simulink model "gm_HFMA_4B_1_5_9_13"  (R2026b)
settings: Solver=FixedStepDiscrete  StopTime=stopTime  FixedStep=1.953125e-06
PreLoadFcn:
  | load('a_luts.mat')
undefined symbols (not defined in the file or in its folder): Ts
libraries: simulink x202, simulink_need_slupdate x99, hdlsllib x91
(part 8 of 20)

== system gm_HFMA_4B_1_5_9_13/Subsystem/crp_temp_shared3 ==
  in0 : Inport  OutDataTypeStr=fixdt(1,16,15,'DataTypeOverride', 'Off')  PortDimensions=1  SampleTime=1.953125e-06
  in1 : Inport  Port=2  OutDataTypeStr=fixdt(1,16,15,'DataTypeOverride', 'Off')  PortDimensions=1  SampleTime=1.953125e-06
  in2 : Inport  Port=3  OutDataTypeStr=fixdt(1,16,15,'DataTypeOverride', 'Off')  PortDimensions=1  SampleTime=1.953125e-06
  in3 : Inport  Port=4  OutDataTypeStr=fixdt(1,16,15,'DataTypeOverride', 'Off')  PortDimensions=1  SampleTime=1.953125e-06
  in4 : Inport  Port=5  OutDataTypeStr=fixdt(1,16,15,'DataTypeOverride', 'Off')  PortDimensions=1  SampleTime=1.953125e-06
  in5 : Inport  Port=6  OutDataTypeStr=fixdt(1,16,15,'DataTypeOverride', 'Off')  PortDimensions=1  SampleTime=1.953125e-06
  in6 : Inport  Port=7  OutDataTypeStr=fixdt(1,16,15,'DataTypeOverride', 'Off')  PortDimensions=1  SampleTime=1.953125e-06
  in7 : Inport  Port=8  OutDataTypeStr=fixdt(1,16,15,'DataTypeOverride', 'Off')  PortDimensions=1  SampleTime=1.953125e-06
  in8 : Inport  Port=9  OutDataTypeStr=fixdt(1,16,15,'DataTypeOverride', 'Off')  PortDimensions=1  SampleTime=1.953125e-06
  in9 : Inport  Port=10  OutDataTypeStr=fixdt(1,16,15,'DataTypeOverride', 'Off')  PortDimensions=1  SampleTime=1.953125e-06
  in10 : Inport  Port=11  OutDataTypeStr=fixdt(1,16,15,'DataTypeOverride', 'Off')  PortDimensions=1  SampleTime=1.953125e-06
  in11 : Inport  Port=12  OutDataTypeStr=fixdt(1,16,15,'DataTypeOverride', 'Off')  PortDimensions=1  SampleTime=1.953125e-06
  in12 : Inport  Port=13  OutDataTypeStr=fixdt(1,16,15,'DataTypeOverride', 'Off')  PortDimensions=1  SampleTime=1.953125e-06
  in13 : Inport  Port=14  OutDataTypeStr=fixdt(1,16,15,'DataTypeOverride', 'Off')  PortDimensions=1  SampleTime=1.953125e-06
  in14 : Inport  Port=15  OutDataTypeStr=fixdt(1,16,15,'DataTypeOverride', 'Off')  PortDimensions=1  SampleTime=1.953125e-06
  in15 : Inport  Port=16  OutDataTypeStr=fixdt(1,16,15,'DataTypeOverride', 'Off')  PortDimensions=1  SampleTime=1.953125e-06
  enb_counter : Inport  Port=17  OutDataTypeStr=fixdt(0,6,0,'DataTypeOverride', 'Off')  PortDimensions=1  SampleTime=1.953125e-06
  Gain1 : Product  Inputs=**  OutDataTypeStr=fixdt(1, 35, 0)  SampleTime=1.953125e-06
  Gain11_const : Constant  Value=0.068999767303466796875  OutDataTypeStr=fixdt(0, 18, 21)  SampleTime=1.953125e-06
  Gain12_const : Constant  Value=0.773799896240234375  OutDataTypeStr=fixdt(0, 18, 18)  SampleTime=1.953125e-06
  Gain13_const : Constant  Value=0.068999767303466796875  OutDataTypeStr=fixdt(0, 18, 21)  SampleTime=1.953125e-06
  Gain14_const : Constant  Value=-0.1882991790771484375  OutDataTypeStr=fixdt(1, 18, 19)  SampleTime=1.953125e-06
  Gain15_const : Constant  Value=0.03100001811981201171875  OutDataTypeStr=fixdt(0, 18, 23)  SampleTime=1.953125e-06
  Gain16_const : Constant  Value=-0.107700347900390625  OutDataTypeStr=fixdt(1, 18, 20)  SampleTime=1.953125e-06
  Gain17_const : Constant  Value=-0.0090999603271484375  OutDataTypeStr=fixdt(1, 18, 23)  SampleTime=1.953125e-06
  Gain18_const : Constant  Value=-0.0370998382568359375  OutDataTypeStr=fixdt(1, 18, 21)  SampleTime=1.953125e-06
  Gain19_const : Constant  Value=-0.0220000743865966796875  OutDataTypeStr=fixdt(1, 18, 22)  SampleTime=1.953125e-06
  Gain1_const : Constant  Value=-0.003899991512298583984375  OutDataTypeStr=fixdt(1, 18, 25)  SampleTime=1.953125e-06
  Gain20_const : Constant  Value=-0.004499971866607666015625  OutDataTypeStr=fixdt(1, 18, 24)  SampleTime=1.953125e-06
  Gain21_const : Constant  Value=-0.0132000446319580078125  OutDataTypeStr=fixdt(1, 18, 23)  SampleTime=1.953125e-06
  Gain22_const : Constant  Value=0.001299999654293060302734375  OutDataTypeStr=fixdt(0, 18, 27)  SampleTime=1.953125e-06
  Gain23_const : Constant  Value=-0.003899991512298583984375  OutDataTypeStr=fixdt(1, 18, 25)  SampleTime=1.953125e-06
  Gain24_const : Constant  Value=0.0005999989807605743408203125  OutDataTypeStr=fixdt(0, 18, 28)  SampleTime=1.953125e-06
  Gain_const : Constant  Value=0.0005999989807605743408203125  OutDataTypeStr=fixdt(0, 18, 28)  SampleTime=1.953125e-06
  Serializer_Subnetwork : Subsystem
  Serializer_Subnetwork1 : Subsystem
  counter : Subsystem
  demux : Demux  Outputs=16
  enb_counter_eq_15 : simulink/Logic and Bit Operations/Compare To Constant  relop===  const=15  OutDataTypeStr=boolean
  enb_counter_le_15 : simulink/Logic and Bit Operations/Compare To Constant  relop=<=  const=15  OutDataTypeStr=boolean
  mux : Mux  Inputs=16
  mux1 : Mux  Inputs=16
  nequ_dtc{,1..15} (16 alike) : DataTypeConversion  OutDataTypeStr=fixdt(1, 19, 0)  ConvertRealWorld=Stored Integer (SI)  SampleTime=1.953125e-06  SaturateOnIntegerOverflow=off  RndMeth=Floor
  nequ_dtc{16..31} (16 alike) : DataTypeConversion  OutDataTypeStr=fixdt(1, 17, 0)  ConvertRealWorld=Stored Integer (SI)  SampleTime=1.953125e-06  SaturateOnIntegerOverflow=off  RndMeth=Floor
  nequ_dtc32 : DataTypeConversion  OutDataTypeStr=fixdt(1, 34, 40)  ConvertRealWorld=Stored Integer (SI)  SampleTime=1.953125e-06  SaturateOnIntegerOverflow=off  RndMeth=Floor
  nequ_dtc33 : DataTypeConversion  OutDataTypeStr=fixdt(1, 34, 43)  ConvertRealWorld=Stored Integer (SI)  SampleTime=1.953125e-06  SaturateOnIntegerOverflow=off  RndMeth=Floor
  nequ_dtc34 : DataTypeConversion  OutDataTypeStr=fixdt(1, 34, 43)  ConvertRealWorld=Stored Integer (SI)  SampleTime=1.953125e-06  SaturateOnIntegerOverflow=off  RndMeth=Floor
  nequ_dtc35 : DataTypeConversion  OutDataTypeStr=fixdt(1, 34, 40)  ConvertRealWorld=Stored Integer (SI)  SampleTime=1.953125e-06  SaturateOnIntegerOverflow=off  RndMeth=Floor
  nequ_dtc36 : DataTypeConversion  OutDataTypeStr=fixdt(1, 34, 42)  ConvertRealWorld=Stored Integer (SI)  SampleTime=1.953125e-06  SaturateOnIntegerOverflow=off  RndMeth=Floor
  nequ_dtc37 : DataTypeConversion  OutDataTypeStr=fixdt(1, 34, 38)  ConvertRealWorld=Stored Integer (SI)  SampleTime=1.953125e-06  SaturateOnIntegerOverflow=off  RndMeth=Floor
  nequ_dtc38 : DataTypeConversion  OutDataTypeStr=fixdt(1, 34, 39)  ConvertRealWorld=Stored Integer (SI)  SampleTime=1.953125e-06  SaturateOnIntegerOverflow=off  RndMeth=Floor
  nequ_dtc39 : DataTypeConversion  OutDataTypeStr=fixdt(1, 34, 37)  ConvertRealWorld=Stored Integer (SI)  SampleTime=1.953125e-06  SaturateOnIntegerOverflow=off  RndMeth=Floor
  nequ_dtc40 : DataTypeConversion  OutDataTypeStr=fixdt(1, 34, 36)  ConvertRealWorld=Stored Integer (SI)  SampleTime=1.953125e-06  SaturateOnIntegerOverflow=off  RndMeth=Floor
  nequ_dtc41 : DataTypeConversion  OutDataTypeStr=fixdt(1, 34, 38)  ConvertRealWorld=Stored Integer (SI)  SampleTime=1.953125e-06  SaturateOnIntegerOverflow=off  RndMeth=Floor
  nequ_dtc42 : DataTypeConversion  OutDataTypeStr=fixdt(1, 34, 35)  ConvertRealWorld=Stored Integer (SI)  SampleTime=1.953125e-06  SaturateOnIntegerOverflow=off  RndMeth=Floor
  nequ_dtc43 : DataTypeConversion  OutDataTypeStr=fixdt(1, 34, 38)  ConvertRealWorld=Stored Integer (SI)  SampleTime=1.953125e-06  SaturateOnIntegerOverflow=off  RndMeth=Floor
  nequ_dtc44 : DataTypeConversion  OutDataTypeStr=fixdt(1, 34, 34)  ConvertRealWorld=Stored Integer (SI)  SampleTime=1.953125e-06  SaturateOnIntegerOverflow=off  RndMeth=Floor
  nequ_dtc45 : DataTypeConversion  OutDataTypeStr=fixdt(1, 34, 36)  ConvertRealWorld=Stored Integer (SI)  SampleTime=1.953125e-06  SaturateOnIntegerOverflow=off  RndMeth=Floor
  nequ_dtc46 : DataTypeConversion  OutDataTypeStr=fixdt(1, 34, 33)  ConvertRealWorld=Stored Integer (SI)  SampleTime=1.953125e-06  SaturateOnIntegerOverflow=off  RndMeth=Floor
  nequ_dtc47 : DataTypeConversion  OutDataTypeStr=fixdt(1, 34, 36)  ConvertRealWorld=Stored Integer (SI)  SampleTime=1.953125e-06  SaturateOnIntegerOverflow=off  RndMeth=Floor
  tapped_delay : hdlsllib/Discrete/Tapped Delay Enabled Synchronous  vinit=0  samptime=-1  NumDelays=15  DelayOrder=Oldest  includeCurrent=on
  tapped_delay_outunit_delay : simulink_need_slupdate/Unit Delay Enabled  vinit=0.0  tsamp=-1
  out0 : Outport  OutDataTypeStr=fixdt(1,34,40,'DataTypeOverride', 'Off')  PortDimensions=1  SampleTime=1.953125e-06
  out1 : Outport  Port=2  OutDataTypeStr=fixdt(1,34,43,'DataTypeOverride', 'Off')  PortDimensions=1  SampleTime=1.953125e-06
  out2 : Outport  Port=3  OutDataTypeStr=fixdt(1,34,43,'DataTypeOverride', 'Off')  PortDimensions=1  SampleTime=1.953125e-06
  out3 : Outport  Port=4  OutDataTypeStr=fixdt(1,34,40,'DataTypeOverride', 'Off')  PortDimensions=1  SampleTime=1.953125e-06
  out4 : Outport  Port=5  OutDataTypeStr=fixdt(1,34,42,'DataTypeOverride', 'Off')  PortDimensions=1  SampleTime=1.953125e-06
  out5 : Outport  Port=6  OutDataTypeStr=fixdt(1,34,38,'DataTypeOverride', 'Off')  PortDimensions=1  SampleTime=1.953125e-06
  out6 : Outport  Port=7  OutDataTypeStr=fixdt(1,34,39,'DataTypeOverride', 'Off')  PortDimensions=1  SampleTime=1.953125e-06
  out7 : Outport  Port=8  OutDataTypeStr=fixdt(1,34,37,'DataTypeOverride', 'Off')  PortDimensions=1  SampleTime=1.953125e-06
  out8 : Outport  Port=9  OutDataTypeStr=fixdt(1,34,36,'DataTypeOverride', 'Off')  PortDimensions=1  SampleTime=1.953125e-06
  out9 : Outport  Port=10  OutDataTypeStr=fixdt(1,34,38,'DataTypeOverride', 'Off')  PortDimensions=1  SampleTime=1.953125e-06
  out10 : Outport  Port=11  OutDataTypeStr=fixdt(1,34,35,'DataTypeOverride', 'Off')  PortDimensions=1  SampleTime=1.953125e-06
  out11 : Outport  Port=12  OutDataTypeStr=fixdt(1,34,38,'DataTypeOverride', 'Off')  PortDimensions=1  SampleTime=1.953125e-06
  out12 : Outport  Port=13  OutDataTypeStr=fixdt(1,34,34,'DataTypeOverride', 'Off')  PortDimensions=1  SampleTime=1.953125e-06
  out13 : Outport  Port=14  OutDataTypeStr=fixdt(1,34,36,'DataTypeOverride', 'Off')  PortDimensions=1  SampleTime=1.953125e-06
  out14 : Outport  Port=15  OutDataTypeStr=fixdt(1,34,33,'DataTypeOverride', 'Off')  PortDimensions=1  SampleTime=1.953125e-06
  out15 : Outport  Port=16  OutDataTypeStr=fixdt(1,34,36,'DataTypeOverride', 'Off')  PortDimensions=1  SampleTime=1.953125e-06
  wires:
  Gain_const/1 -> nequ_dtc1/1
  Gain1/1 -> tapped_delay/1
  Gain23_const/1 -> nequ_dtc3/1
  nequ_dtc47/1 -> out15/1
  Gain1_const/1 -> nequ_dtc/1
  Gain24_const/1 -> nequ_dtc2/1
  nequ_dtc18/1 -> mux1/3
  Gain22_const/1 -> nequ_dtc4/1
  Gain20_const/1 -> nequ_dtc6/1
  Gain21_const/1 -> nequ_dtc5/1
  Gain13_const/1 -> nequ_dtc13/1
  Gain15_const/1 -> nequ_dtc11/1
  Gain17_const/1 -> nequ_dtc9/1
  Gain19_const/1 -> nequ_dtc7/1
  Gain12_const/1 -> nequ_dtc14/1
  Gain14_const/1 -> nequ_dtc12/1
  Gain16_const/1 -> nequ_dtc10/1
  Gain18_const/1 -> nequ_dtc8/1
  Gain11_const/1 -> nequ_dtc15/1
  nequ_dtc42/1 -> out10/1
  in0/1 -> nequ_dtc16/1
  nequ_dtc43/1 -> out11/1
  in1/1 -> nequ_dtc17/1
  in6/1 -> nequ_dtc22/1
  in2/1 -> nequ_dtc18/1
  in3/1 -> nequ_dtc19/1
  in4/1 -> nequ_dtc20/1
  nequ_dtc39/1 -> out7/1
  in5/1 -> nequ_dtc21/1
  in11/1 -> nequ_dtc27/1
  in7/1 -> nequ_dtc23/1
  demux/13 -> nequ_dtc44/1
  in12/1 -> nequ_dtc28/1
  demux/9 -> nequ_dtc40/1
  in8/1 -> nequ_dtc24/1
  demux/12 -> nequ_dtc43/1
  in9/1 -> nequ_dtc25/1
  in10/1 -> nequ_dtc26/1
  in13/1 -> nequ_dtc29/1
  nequ_dtc30/1 -> mux1/15
  demux/7 -> nequ_dtc38/1
  in14/1 -> nequ_dtc30/1
  in15/1 -> nequ_dtc31/1
  demux/1 -> nequ_dtc32/1
  enb_counter/1 -> enb_counter_eq_15/1, enb_counter_le_15/1
  nequ_dtc/1 -> mux/1
  nequ_dtc1/1 -> mux/2
  nequ_dtc2/1 -> mux/3
  nequ_dtc3/1 -> mux/4
  nequ_dtc8/1 -> mux/9
  nequ_dtc4/1 -> mux/5
  nequ_dtc5/1 -> mux/6
  nequ_dtc6/1 -> mux/7
  nequ_dtc7/1 -> mux/8
  nequ_dtc13/1 -> mux/14
  nequ_dtc9/1 -> mux/10
  nequ_dtc10/1 -> mux/11
  nequ_dtc11/1 -> mux/12
  nequ_dtc12/1 -> mux/13
  nequ_dtc14/1 -> mux/15
  nequ_dtc15/1 -> mux/16
  nequ_dtc16/1 -> mux1/1
  nequ_dtc17/1 -> mux1/2
  nequ_dtc23/1 -> mux1/8
  nequ_dtc19/1 -> mux1/4
  nequ_dtc20/1 -> mux1/5
  nequ_dtc21/1 -> mux1/6
  nequ_dtc22/1 -> mux1/7
  nequ_dtc28/1 -> mux1/13
  nequ_dtc24/1 -> mux1/9
  nequ_dtc29/1 -> mux1/14
  nequ_dtc25/1 -> mux1/10
  nequ_dtc26/1 -> mux1/11
  nequ_dtc27/1 -> mux1/12
  nequ_dtc31/1 -> mux1/16
  enb_counter_le_15/1 -> counter/Enable, tapped_delay/2
  mux/1 -> Serializer_Subnetwork/1(in0)
  mux1/1 -> Serializer_Subnetwork1/1(in0)
  counter/1(out0) -> Serializer_Subnetwork1/2(in1), Serializer_Subnetwork/2(in1)
  Serializer_Subnetwork/1(out0) -> Gain1/1
  demux/2 -> nequ_dtc33/1
  Serializer_Subnetwork1/1(out0) -> Gain1/2
  enb_counter_eq_15/1 -> tapped_delay_outunit_delay/2
  tapped_delay/1 -> tapped_delay_outunit_delay/1
  tapped_delay_outunit_delay/1 -> demux/1
  demux/3 -> nequ_dtc34/1
  demux/4 -> nequ_dtc35/1
  demux/5 -> nequ_dtc36/1
  demux/6 -> nequ_dtc37/1
  demux/8 -> nequ_dtc39/1
  demux/10 -> nequ_dtc41/1
  demux/11 -> nequ_dtc42/1
  demux/14 -> nequ_dtc45/1
  demux/15 -> nequ_dtc46/1
  demux/16 -> nequ_dtc47/1
  nequ_dtc32/1 -> out0/1
  nequ_dtc33/1 -> out1/1
  nequ_dtc34/1 -> out2/1
  nequ_dtc35/1 -> out3/1
  nequ_dtc36/1 -> out4/1
  nequ_dtc37/1 -> out5/1
  nequ_dtc38/1 -> out6/1
  nequ_dtc40/1 -> out8/1
  nequ_dtc41/1 -> out9/1
  nequ_dtc44/1 -> out12/1
  nequ_dtc45/1 -> out13/1
  nequ_dtc46/1 -> out14/1

== system gm_HFMA_4B_1_5_9_13/Subsystem/crp_temp_shared4 ==
  in0 : Inport  OutDataTypeStr=fixdt(1,16,15,'DataTypeOverride', 'Off')  PortDimensions=1  SampleTime=1.953125e-06
  in1 : Inport  Port=2  OutDataTypeStr=fixdt(1,16,15,'DataTypeOverride', 'Off')  PortDimensions=1  SampleTime=1.953125e-06
  in2 : Inport  Port=3  OutDataTypeStr=fixdt(1,16,15,'DataTypeOverride', 'Off')  PortDimensions=1  SampleTime=1.953125e-06
  in3 : Inport  Port=4  OutDataTypeStr=fixdt(1,16,15,'DataTypeOverride', 'Off')  PortDimensions=1  SampleTime=1.953125e-06
  in4 : Inport  Port=5  OutDataTypeStr=fixdt(1,16,15,'DataTypeOverride', 'Off')  PortDimensions=1  SampleTime=1.953125e-06
  in5 : Inport  Port=6  OutDataTypeStr=fixdt(1,16,15,'DataTypeOverride', 'Off')  PortDimensions=1  SampleTime=1.953125e-06
  in6 : Inport  Port=7  OutDataTypeStr=fixdt(1,16,15,'DataTypeOverride', 'Off')  PortDimensions=1  SampleTime=1.953125e-06
  in7 : Inport  Port=8  OutDataTypeStr=fixdt(1,16,15,'DataTypeOverride', 'Off')  PortDimensions=1  SampleTime=1.953125e-06
  in8 : Inport  Port=9  OutDataTypeStr=fixdt(1,16,15,'DataTypeOverride', 'Off')  PortDimensions=1  SampleTime=1.953125e-06
  in9 : Inport  Port=10  OutDataTypeStr=fixdt(1,16,15,'DataTypeOverride', 'Off')  PortDimensions=1  SampleTime=1.953125e-06
  in10 : Inport  Port=11  OutDataTypeStr=fixdt(1,16,15,'DataTypeOverride', 'Off')  PortDimensions=1  SampleTime=1.953125e-06
  in11 : Inport  Port=12  OutDataTypeStr=fixdt(1,16,15,'DataTypeOverride', 'Off')  PortDimensions=1  SampleTime=1.953125e-06
  in12 : Inport  Port=13  OutDataTypeStr=fixdt(1,16,15,'DataTypeOverride', 'Off')  PortDimensions=1  SampleTime=1.953125e-06
  in13 : Inport  Port=14  OutDataTypeStr=fixdt(1,16,15,'DataTypeOverride', 'Off')  PortDimensions=1  SampleTime=1.953125e-06
  in14 : Inport  Port=15  OutDataTypeStr=fixdt(1,16,15,'DataTypeOverride', 'Off')  PortDimensions=1  SampleTime=1.953125e-06
  in15 : Inport  Port=16  OutDataTypeStr=fixdt(1,16,15,'DataTypeOverride', 'Off')  PortDimensions=1  SampleTime=1.953125e-06
  enb_counter : Inport  Port=17  OutDataTypeStr=fixdt(0,6,0,'DataTypeOverride', 'Off')  PortDimensions=1  SampleTime=1.953125e-06
  Gain10 : Product  Inputs=**  OutDataTypeStr=fixdt(1, 35, 0)  SampleTime=1.953125e-06
  Gain10_const : Constant  Value=-0.1882991790771484375  OutDataTypeStr=fixdt(1, 18, 19)  SampleTime=1.953125e-06
  Gain1_const : Constant  Value=-0.003899991512298583984375  OutDataTypeStr=fixdt(1, 18, 25)  SampleTime=1.953125e-06
  Gain20_const : Constant  Value=-0.004499971866607666015625  OutDataTypeStr=fixdt(1, 18, 24)  SampleTime=1.953125e-06
  Gain21_const : Constant  Value=-0.0132000446319580078125  OutDataTypeStr=fixdt(1, 18, 23)  SampleTime=1.953125e-06
  Gain22_const : Constant  Value=0.001299999654293060302734375  OutDataTypeStr=fixdt(0, 18, 27)  SampleTime=1.953125e-06
  Gain23_const : Constant  Value=-0.003899991512298583984375  OutDataTypeStr=fixdt(1, 18, 25)  SampleTime=1.953125e-06
  Gain24_const : Constant  Value=0.0005999989807605743408203125  OutDataTypeStr=fixdt(0, 18, 28)  SampleTime=1.953125e-06
  Gain2_const : Constant  Value=0.001299999654293060302734375  OutDataTypeStr=fixdt(0, 18, 27)  SampleTime=1.953125e-06
  Gain3_const : Constant  Value=-0.0132000446319580078125  OutDataTypeStr=fixdt(1, 18, 23)  SampleTime=1.953125e-06
  Gain4_const : Constant  Value=-0.004499971866607666015625  OutDataTypeStr=fixdt(1, 18, 24)  SampleTime=1.953125e-06
  Gain5_const : Constant  Value=-0.0220000743865966796875  OutDataTypeStr=fixdt(1, 18, 22)  SampleTime=1.953125e-06
  Gain6_const : Constant  Value=-0.0370998382568359375  OutDataTypeStr=fixdt(1, 18, 21)  SampleTime=1.953125e-06
  Gain7_const : Constant  Value=-0.0090999603271484375  OutDataTypeStr=fixdt(1, 18, 23)  SampleTime=1.953125e-06
  Gain8_const : Constant  Value=-0.107700347900390625  OutDataTypeStr=fixdt(1, 18, 20)  SampleTime=1.953125e-06
  Gain9_const : Constant  Value=0.03100001811981201171875  OutDataTypeStr=fixdt(0, 18, 23)  SampleTime=1.953125e-06
  Gain_const : Constant  Value=0.0005999989807605743408203125  OutDataTypeStr=fixdt(0, 18, 28)  SampleTime=1.953125e-06
  Serializer_Subnetwork : Subsystem
  Serializer_Subnetwork1 : Subsystem
  counter : Subsystem
  demux : Demux  Outputs=16
  enb_counter_eq_15 : simulink/Logic and Bit Operations/Compare To Constant  relop===  const=15  OutDataTypeStr=boolean
  enb_counter_le_15 : simulink/Logic and Bit Operations/Compare To Constant  relop=<=  const=15  OutDataTypeStr=boolean
  mux : Mux  Inputs=16
  mux1 : Mux  Inputs=16
  nequ_dtc{,1..15} (16 alike) : DataTypeConversion  OutDataTypeStr=fixdt(1, 19, 0)  ConvertRealWorld=Stored Integer (SI)  SampleTime=1.953125e-06  SaturateOnIntegerOverflow=off  RndMeth=Floor
  nequ_dtc{16..31} (16 alike) : DataTypeConversion  OutDataTypeStr=fixdt(1, 17, 0)  ConvertRealWorld=Stored Integer (SI)  SampleTime=1.953125e-06  SaturateOnIntegerOverflow=off  RndMeth=Floor
  nequ_dtc32 : DataTypeConversion  OutDataTypeStr=fixdt(1, 34, 34)  ConvertRealWorld=Stored Integer (SI)  SampleTime=1.953125e-06  SaturateOnIntegerOverflow=off  RndMeth=Floor
  nequ_dtc{33,35,39,46} (4 alike) : DataTypeConversion  OutDataTypeStr=fixdt(1, 34, 38)  ConvertRealWorld=Stored Integer (SI)  SampleTime=1.953125e-06  SaturateOnIntegerOverflow=off  RndMeth=Floor
  nequ_dtc34 : DataTypeConversion  OutDataTypeStr=fixdt(1, 34, 35)  ConvertRealWorld=Stored Integer (SI)  SampleTime=1.953125e-06  SaturateOnIntegerOverflow=off  RndMeth=Floor
  nequ_dtc36 : DataTypeConversion  OutDataTypeStr=fixdt(1, 34, 36)  ConvertRealWorld=Stored Integer (SI)  SampleTime=1.953125e-06  SaturateOnIntegerOverflow=off  RndMeth=Floor
  nequ_dtc37 : DataTypeConversion  OutDataTypeStr=fixdt(1, 34, 37)  ConvertRealWorld=Stored Integer (SI)  SampleTime=1.953125e-06  SaturateOnIntegerOverflow=off  RndMeth=Floor
  nequ_dtc38 : DataTypeConversion  OutDataTypeStr=fixdt(1, 34, 39)  ConvertRealWorld=Stored Integer (SI)  SampleTime=1.953125e-06  SaturateOnIntegerOverflow=off  RndMeth=Floor
  nequ_dtc40 : DataTypeConversion  OutDataTypeStr=fixdt(1, 34, 42)  ConvertRealWorld=Stored Integer (SI)  SampleTime=1.953125e-06  SaturateOnIntegerOverflow=off  RndMeth=Floor
  nequ_dtc41 : DataTypeConversion  OutDataTypeStr=fixdt(1, 34, 40)  ConvertRealWorld=Stored Integer (SI)  SampleTime=1.953125e-06  SaturateOnIntegerOverflow=off  RndMeth=Floor
  nequ_dtc42 : DataTypeConversion  OutDataTypeStr=fixdt(1, 34, 43)  ConvertRealWorld=Stored Integer (SI)  SampleTime=1.953125e-06  SaturateOnIntegerOverflow=off  RndMeth=Floor
  nequ_dtc43 : DataTypeConversion  OutDataTypeStr=fixdt(1, 34, 43)  ConvertRealWorld=Stored Integer (SI)  SampleTime=1.953125e-06  SaturateOnIntegerOverflow=off  RndMeth=Floor
  nequ_dtc44 : DataTypeConversion  OutDataTypeStr=fixdt(1, 34, 40)  ConvertRealWorld=Stored Integer (SI)  SampleTime=1.953125e-06  SaturateOnIntegerOverflow=off  RndMeth=Floor
  nequ_dtc45 : DataTypeConversion  OutDataTypeStr=fixdt(1, 34, 42)  ConvertRealWorld=Stored Integer (SI)  SampleTime=1.953125e-06  SaturateOnIntegerOverflow=off  RndMeth=Floor
  nequ_dtc47 : DataTypeConversion  OutDataTypeStr=fixdt(1, 34, 39)  ConvertRealWorld=Stored Integer (SI)  SampleTime=1.953125e-06  SaturateOnIntegerOverflow=off  RndMeth=Floor
  tapped_delay : hdlsllib/Discrete/Tapped Delay Enabled Synchronous  vinit=0  samptime=-1  NumDelays=15  DelayOrder=Oldest  includeCurrent=on
  tapped_delay_outunit_delay : simulink_need_slupdate/Unit Delay Enabled  vinit=0.0  tsamp=-1
  out0 : Outport  OutDataTypeStr=fixdt(1,34,34,'DataTypeOverride', 'Off')  PortDimensions=1  SampleTime=1.953125e-06
  out1 : Outport  Port=2  OutDataTypeStr=fixdt(1,34,38,'DataTypeOverride', 'Off')  PortDimensions=1  SampleTime=1.953125e-06
  out2 : Outport  Port=3  OutDataTypeStr=fixdt(1,34,35,'DataTypeOverride', 'Off')  PortDimensions=1  SampleTime=1.953125e-06
  out3 : Outport  Port=4  OutDataTypeStr=fixdt(1,34,38,'DataTypeOverride', 'Off')  PortDimensions=1  SampleTime=1.953125e-06
  out4 : Outport  Port=5  OutDataTypeStr=fixdt(1,34,36,'DataTypeOverride', 'Off')  PortDimensions=1  SampleTime=1.953125e-06
  out5 : Outport  Port=6  OutDataTypeStr=fixdt(1,34,37,'DataTypeOverride', 'Off')  PortDimensions=1  SampleTime=1.953125e-06
  out6 : Outport  Port=7  OutDataTypeStr=fixdt(1,34,39,'DataTypeOverride', 'Off')  PortDimensions=1  SampleTime=1.953125e-06
  out7 : Outport  Port=8  OutDataTypeStr=fixdt(1,34,38,'DataTypeOverride', 'Off')  PortDimensions=1  SampleTime=1.953125e-06
  out8 : Outport  Port=9  OutDataTypeStr=fixdt(1,34,42,'DataTypeOverride', 'Off')  PortDimensions=1  SampleTime=1.953125e-06
  out9 : Outport  Port=10  OutDataTypeStr=fixdt(1,34,40,'DataTypeOverride', 'Off')  PortDimensions=1  SampleTime=1.953125e-06
  out10 : Outport  Port=11  OutDataTypeStr=fixdt(1,34,43,'DataTypeOverride', 'Off')  PortDimensions=1  SampleTime=1.953125e-06
  out11 : Outport  Port=12  OutDataTypeStr=fixdt(1,34,43,'DataTypeOverride', 'Off')  PortDimensions=1  SampleTime=1.953125e-06
  out12 : Outport  Port=13  OutDataTypeStr=fixdt(1,34,40,'DataTypeOverride', 'Off')  PortDimensions=1  SampleTime=1.953125e-06
  out13 : Outport  Port=14  OutDataTypeStr=fixdt(1,34,42,'DataTypeOverride', 'Off')  PortDimensions=1  SampleTime=1.953125e-06
  out14 : Outport  Port=15  OutDataTypeStr=fixdt(1,34,38,'DataTypeOverride', 'Off')  PortDimensions=1  SampleTime=1.953125e-06
  out15 : Outport  Port=16  OutDataTypeStr=fixdt(1,34,39,'DataTypeOverride', 'Off')  PortDimensions=1  SampleTime=1.953125e-06
  wires:
  Gain6_const/1 -> nequ_dtc4/1
  nequ_dtc30/1 -> mux1/15
  Gain9_const/1 -> nequ_dtc1/1
  Gain10/1 -> tapped_delay/1
  Gain7_const/1 -> nequ_dtc3/1
  Gain10_const/1 -> nequ_dtc/1
  Gain8_const/1 -> nequ_dtc2/1
  Gain24_const/1 -> nequ_dtc11/1
  Gain1_const/1 -> nequ_dtc9/1
  Gain5_const/1 -> nequ_dtc5/1
  Gain3_const/1 -> nequ_dtc7/1
  Gain_const/1 -> nequ_dtc10/1
  Gain2_const/1 -> nequ_dtc8/1
  Gain4_const/1 -> nequ_dtc6/1
  Gain21_const/1 -> nequ_dtc14/1
  Gain23_const/1 -> nequ_dtc12/1
  Gain20_const/1 -> nequ_dtc15/1
  Gain22_const/1 -> nequ_dtc13/1
  nequ_dtc19/1 -> mux1/4
  in4/1 -> nequ_dtc20/1
  in0/1 -> nequ_dtc16/1
  in5/1 -> nequ_dtc21/1
  nequ_dtc22/1 -> mux1/7
  nequ_dtc18/1 -> mux1/3
  in1/1 -> nequ_dtc17/1
  nequ_dtc21/1 -> mux1/6
  nequ_dtc17/1 -> mux1/2
  in2/1 -> nequ_dtc18/1
  nequ_dtc20/1 -> mux1/5
  in3/1 -> nequ_dtc19/1
  in10/1 -> nequ_dtc26/1
  in6/1 -> nequ_dtc22/1
  in7/1 -> nequ_dtc23/1
  in8/1 -> nequ_dtc24/1
  in9/1 -> nequ_dtc25/1
  in15/1 -> nequ_dtc31/1
  in11/1 -> nequ_dtc27/1
  in12/1 -> nequ_dtc28/1
  in13/1 -> nequ_dtc29/1
  in14/1 -> nequ_dtc30/1
  enb_counter/1 -> enb_counter_eq_15/1, enb_counter_le_15/1
  nequ_dtc/1 -> mux/1
  nequ_dtc1/1 -> mux/2
  nequ_dtc6/1 -> mux/7
  nequ_dtc2/1 -> mux/3
  nequ_dtc3/1 -> mux/4
  nequ_dtc4/1 -> mux/5
  nequ_dtc5/1 -> mux/6
  nequ_dtc11/1 -> mux/12
  nequ_dtc7/1 -> mux/8
  nequ_dtc12/1 -> mux/13
  nequ_dtc8/1 -> mux/9
  nequ_dtc9/1 -> mux/10
  nequ_dtc10/1 -> mux/11
  nequ_dtc13/1 -> mux/14
  nequ_dtc14/1 -> mux/15
  nequ_dtc15/1 -> mux/16
  nequ_dtc16/1 -> mux1/1
  nequ_dtc27/1 -> mux1/12
  nequ_dtc23/1 -> mux1/8
  nequ_dtc24/1 -> mux1/9
  nequ_dtc25/1 -> mux1/10
  nequ_dtc26/1 -> mux1/11
  nequ_dtc28/1 -> mux1/13
  nequ_dtc29/1 -> mux1/14
  nequ_dtc31/1 -> mux1/16
  enb_counter_le_15/1 -> counter/Enable, tapped_delay/2
  mux/1 -> Serializer_Subnetwork/1(in0)
  mux1/1 -> Serializer_Subnetwork1/1(in0)
  counter/1(out0) -> Serializer_Subnetwork1/2(in1), Serializer_Subnetwork/2(in1)
  Serializer_Subnetwork/1(out0) -> Gain10/1
  Serializer_Subnetwork1/1(out0) -> Gain10/2
  enb_counter_eq_15/1 -> tapped_delay_outunit_delay/2
  tapped_delay/1 -> tapped_delay_outunit_delay/1
  tapped_delay_outunit_delay/1 -> demux/1
  demux/1 -> nequ_dtc32/1
  demux/2 -> nequ_dtc33/1
  demux/3 -> nequ_dtc34/1
  demux/4 -> nequ_dtc35/1
  demux/5 -> nequ_dtc36/1
  demux/6 -> nequ_dtc37/1
  demux/7 -> nequ_dtc38/1
  demux/8 -> nequ_dtc39/1
  demux/9 -> nequ_dtc40/1
  demux/10 -> nequ_dtc41/1
  demux/11 -> nequ_dtc42/1
  demux/12 -> nequ_dtc43/1
  demux/13 -> nequ_dtc44/1
  demux/14 -> nequ_dtc45/1
  demux/15 -> nequ_dtc46/1
  demux/16 -> nequ_dtc47/1
  nequ_dtc32/1 -> out0/1
  nequ_dtc33/1 -> out1/1
  nequ_dtc34/1 -> out2/1
  nequ_dtc35/1 -> out3/1
  nequ_dtc36/1 -> out4/1
  nequ_dtc37/1 -> out5/1
  nequ_dtc38/1 -> out6/1
  nequ_dtc39/1 -> out7/1
  nequ_dtc40/1 -> out8/1
  nequ_dtc41/1 -> out9/1
  nequ_dtc42/1 -> out10/1
  nequ_dtc43/1 -> out11/1
  nequ_dtc44/1 -> out12/1
  nequ_dtc45/1 -> out13/1
  nequ_dtc46/1 -> out14/1
  nequ_dtc47/1 -> out15/1

== system gm_HFMA_4B_1_5_9_13/Subsystem/crp_temp_shared5 ==
  in0 : Inport  OutDataTypeStr=fixdt(1,16,15,'DataTypeOverride', 'Off')  PortDimensions=1  SampleTime=1.953125e-06
  in1 : Inport  Port=2  OutDataTypeStr=fixdt(1,16,15,'DataTypeOverride', 'Off')  PortDimensions=1  SampleTime=1.953125e-06
  in2 : Inport  Port=3  OutDataTypeStr=fixdt(1,16,15,'DataTypeOverride', 'Off')  PortDimensions=1  SampleTime=1.953125e-06
  in3 : Inport  Port=4  OutDataTypeStr=fixdt(1,16,15,'DataTypeOverride', 'Off')  PortDimensions=1  SampleTime=1.953125e-06
  in4 : Inport  Port=5  OutDataTypeStr=fixdt(1,16,15,'DataTypeOverride', 'Off')  PortDimensions=1  SampleTime=1.953125e-06
  in5 : Inport  Port=6  OutDataTypeStr=fixdt(1,16,15,'DataTypeOverride', 'Off')  PortDimensions=1  SampleTime=1.953125e-06
  in6 : Inport  Port=7  OutDataTypeStr=fixdt(1,16,15,'DataTypeOverride', 'Off')  PortDimensions=1  SampleTime=1.953125e-06
  in7 : Inport  Port=8  OutDataTypeStr=fixdt(1,16,15,'DataTypeOverride', 'Off')  PortDimensions=1  SampleTime=1.953125e-06
  in8 : Inport  Port=9  OutDataTypeStr=fixdt(1,16,15,'DataTypeOverride', 'Off')  PortDimensions=1  SampleTime=1.953125e-06
  in9 : Inport  Port=10  OutDataTypeStr=fixdt(1,16,15,'DataTypeOverride', 'Off')  PortDimensions=1  SampleTime=1.953125e-06
  in10 : Inport  Port=11  OutDataTypeStr=fixdt(1,16,15,'DataTypeOverride', 'Off')  PortDimensions=1  SampleTime=1.953125e-06
  in11 : Inport  Port=12  OutDataTypeStr=fixdt(1,16,15,'DataTypeOverride', 'Off')  PortDimensions=1  SampleTime=1.953125e-06
  in12 : Inport  Port=13  OutDataTypeStr=fixdt(1,16,15,'DataTypeOverride', 'Off')  PortDimensions=1  SampleTime=1.953125e-06
  in13 : Inport  Port=14  OutDataTypeStr=fixdt(1,16,15,'DataTypeOverride', 'Off')  PortDimensions=1  SampleTime=1.953125e-06
  in14 : Inport  Port=15  OutDataTypeStr=fixdt(1,16,15,'DataTypeOverride', 'Off')  PortDimensions=1  SampleTime=1.953125e-06
  in15 : Inport  Port=16  OutDataTypeStr=fixdt(1,16,15,'DataTypeOverride', 'Off')  PortDimensions=1  SampleTime=1.953125e-06
  enb_counter : Inport  Port=17  OutDataTypeStr=fixdt(0,6,0,'DataTypeOverride', 'Off')  PortDimensions=1  SampleTime=1.953125e-06
  Gain10_const : Constant  Value=-0.1882991790771484375  OutDataTypeStr=fixdt(1, 18, 19)  SampleTime=1.953125e-06
  Gain11_const : Constant  Value=0.068999767303466796875  OutDataTypeStr=fixdt(0, 18, 21)  SampleTime=1.953125e-06
  Gain12_const : Constant  Value=0.773799896240234375  OutDataTypeStr=fixdt(0, 18, 18)  SampleTime=1.953125e-06
  Gain13_const : Constant  Value=0.068999767303466796875  OutDataTypeStr=fixdt(0, 18, 21)  SampleTime=1.953125e-06
  Gain14_const : Constant  Value=-0.1882991790771484375  OutDataTypeStr=fixdt(1, 18, 19)  SampleTime=1.953125e-06
  Gain15_const : Constant  Value=0.03100001811981201171875  OutDataTypeStr=fixdt(0, 18, 23)  SampleTime=1.953125e-06
  Gain16_const : Constant  Value=-0.107700347900390625  OutDataTypeStr=fixdt(1, 18, 20)  SampleTime=1.953125e-06
  Gain17_const : Constant  Value=-0.0090999603271484375  OutDataTypeStr=fixdt(1, 18, 23)  SampleTime=1.953125e-06
  Gain18_const : Constant  Value=-0.0370998382568359375  OutDataTypeStr=fixdt(1, 18, 21)  SampleTime=1.953125e-06
  Gain19 : Product  Inputs=**  OutDataTypeStr=fixdt(1, 35, 0)  SampleTime=1.953125e-06
  Gain19_const : Constant  Value=-0.0220000743865966796875  OutDataTypeStr=fixdt(1, 18, 22)  SampleTime=1.953125e-06
  Gain4_const : Constant  Value=-0.004499971866607666015625  OutDataTypeStr=fixdt(1, 18, 24)  SampleTime=1.953125e-06
  Gain5_const : Constant  Value=-0.0220000743865966796875  OutDataTypeStr=fixdt(1, 18, 22)  SampleTime=1.953125e-06
  Gain6_const : Constant  Value=-0.0370998382568359375  OutDataTypeStr=fixdt(1, 18, 21)  SampleTime=1.953125e-06
  Gain7_const : Constant  Value=-0.0090999603271484375  OutDataTypeStr=fixdt(1, 18, 23)  SampleTime=1.953125e-06
  Gain8_const : Constant  Value=-0.107700347900390625  OutDataTypeStr=fixdt(1, 18, 20)  SampleTime=1.953125e-06
  Gain9_const : Constant  Value=0.03100001811981201171875  OutDataTypeStr=fixdt(0, 18, 23)  SampleTime=1.953125e-06
  Serializer_Subnetwork : Subsystem
  Serializer_Subnetwork1 : Subsystem
  counter : Subsystem
  demux : Demux  Outputs=16
  enb_counter_eq_15 : simulink/Logic and Bit Operations/Compare To Constant  relop===  const=15  OutDataTypeStr=boolean
  enb_counter_le_15 : simulink/Logic and Bit Operations/Compare To Constant  relop=<=  const=15  OutDataTypeStr=boolean
  mux : Mux  Inputs=16
  mux1 : Mux  Inputs=16
  nequ_dtc{,1..15} (16 alike) : DataTypeConversion  OutDataTypeStr=fixdt(1, 19, 0)  ConvertRealWorld=Stored Integer (SI)  SampleTime=1.953125e-06  SaturateOnIntegerOverflow=off  RndMeth=Floor
  nequ_dtc{16..31} (16 alike) : DataTypeConversion  OutDataTypeStr=fixdt(1, 17, 0)  ConvertRealWorld=Stored Integer (SI)  SampleTime=1.953125e-06  SaturateOnIntegerOverflow=off  RndMeth=Floor
  nequ_dtc32 : DataTypeConversion  OutDataTypeStr=fixdt(1, 34, 37)  ConvertRealWorld=Stored Integer (SI)  SampleTime=1.953125e-06  SaturateOnIntegerOverflow=off  RndMeth=Floor
  nequ_dtc{33,38,40,45} (4 alike) : DataTypeConversion  OutDataTypeStr=fixdt(1, 34, 36)  ConvertRealWorld=Stored Integer (SI)  SampleTime=1.953125e-06  SaturateOnIntegerOverflow=off  RndMeth=Floor
  nequ_dtc{34,36,42,44} (4 alike) : DataTypeConversion  OutDataTypeStr=fixdt(1, 34, 38)  ConvertRealWorld=Stored Integer (SI)  SampleTime=1.953125e-06  SaturateOnIntegerOverflow=off  RndMeth=Floor
  nequ_dtc35 : DataTypeConversion  OutDataTypeStr=fixdt(1, 34, 35)  ConvertRealWorld=Stored Integer (SI)  SampleTime=1.953125e-06  SaturateOnIntegerOverflow=off  RndMeth=Floor
  nequ_dtc37 : DataTypeConversion  OutDataTypeStr=fixdt(1, 34, 34)  ConvertRealWorld=Stored Integer (SI)  SampleTime=1.953125e-06  SaturateOnIntegerOverflow=off  RndMeth=Floor
  nequ_dtc39 : DataTypeConversion  OutDataTypeStr=fixdt(1, 34, 33)  ConvertRealWorld=Stored Integer (SI)  SampleTime=1.953125e-06  SaturateOnIntegerOverflow=off  RndMeth=Floor
  nequ_dtc41 : DataTypeConversion  OutDataTypeStr=fixdt(1, 34, 34)  ConvertRealWorld=Stored Integer (SI)  SampleTime=1.953125e-06  SaturateOnIntegerOverflow=off  RndMeth=Floor
  nequ_dtc43 : DataTypeConversion  OutDataTypeStr=fixdt(1, 34, 35)  ConvertRealWorld=Stored Integer (SI)  SampleTime=1.953125e-06  SaturateOnIntegerOverflow=off  RndMeth=Floor
  nequ_dtc46 : DataTypeConversion  OutDataTypeStr=fixdt(1, 34, 37)  ConvertRealWorld=Stored Integer (SI)  SampleTime=1.953125e-06  SaturateOnIntegerOverflow=off  RndMeth=Floor
  nequ_dtc47 : DataTypeConversion  OutDataTypeStr=fixdt(1, 34, 39)  ConvertRealWorld=Stored Integer (SI)  SampleTime=1.953125e-06  SaturateOnIntegerOverflow=off  RndMeth=Floor
  tapped_delay : hdlsllib/Discrete/Tapped Delay Enabled Synchronous  vinit=0  samptime=-1  NumDelays=15  DelayOrder=Oldest  includeCurrent=on
  tapped_delay_outunit_delay : simulink_need_slupdate/Unit Delay Enabled  vinit=0.0  tsamp=-1
  out0 : Outport  OutDataTypeStr=fixdt(1,34,37,'DataTypeOverride', 'Off')  PortDimensions=1  SampleTime=1.953125e-06
  out1 : Outport  Port=2  OutDataTypeStr=fixdt(1,34,36,'DataTypeOverride', 'Off')  PortDimensions=1  SampleTime=1.953125e-06
  out2 : Outport  Port=3  OutDataTypeStr=fixdt(1,34,38,'DataTypeOverride', 'Off')  PortDimensions=1  SampleTime=1.953125e-06
  out3 : Outport  Port=4  OutDataTypeStr=fixdt(1,34,35,'DataTypeOverride', 'Off')  PortDimensions=1  SampleTime=1.953125e-06
  out4 : Outport  Port=5  OutDataTypeStr=fixdt(1,34,38,'DataTypeOverride', 'Off')  PortDimensions=1  SampleTime=1.953125e-06
  out5 : Outport  Port=6  OutDataTypeStr=fixdt(1,34,34,'DataTypeOverride', 'Off')  PortDimensions=1  SampleTime=1.953125e-06
  out6 : Outport  Port=7  OutDataTypeStr=fixdt(1,34,36,'DataTypeOverride', 'Off')  PortDimensions=1  SampleTime=1.953125e-06
  out7 : Outport  Port=8  OutDataTypeStr=fixdt(1,34,33,'DataTypeOverride', 'Off')  PortDimensions=1  SampleTime=1.953125e-06
  out8 : Outport  Port=9  OutDataTypeStr=fixdt(1,34,36,'DataTypeOverride', 'Off')  PortDimensions=1  SampleTime=1.953125e-06
  out9 : Outport  Port=10  OutDataTypeStr=fixdt(1,34,34,'DataTypeOverride', 'Off')  PortDimensions=1  SampleTime=1.953125e-06
  out10 : Outport  Port=11  OutDataTypeStr=fixdt(1,34,38,'DataTypeOverride', 'Off')  PortDimensions=1  SampleTime=1.953125e-06
  out11 : Outport  Port=12  OutDataTypeStr=fixdt(1,34,35,'DataTypeOverride', 'Off')  PortDimensions=1  SampleTime=1.953125e-06
  out12 : Outport  Port=13  OutDataTypeStr=fixdt(1,34,38,'DataTypeOverride', 'Off')  PortDimensions=1  SampleTime=1.953125e-06
  out13 : Outport  Port=14  OutDataTypeStr=fixdt(1,34,36,'DataTypeOverride', 'Off')  PortDimensions=1  SampleTime=1.953125e-06
  out14 : Outport  Port=15  OutDataTypeStr=fixdt(1,34,37,'DataTypeOverride', 'Off')  PortDimensions=1  SampleTime=1.953125e-06
  out15 : Outport  Port=16  OutDataTypeStr=fixdt(1,34,39,'DataTypeOverride', 'Off')  PortDimensions=1  SampleTime=1.953125e-06
  wires:
  nequ_dtc12/1 -> mux/13
  Gain15_const/1 -> nequ_dtc4/1
  Gain18_const/1 -> nequ_dtc1/1
  Gain19_const/1 -> nequ_dtc/1
  nequ_dtc8/1 -> mux/9
  Gain16_const/1 -> nequ_dtc3/1
  nequ_dtc10/1 -> mux/11
  nequ_dtc6/1 -> mux/7
  Gain17_const/1 -> nequ_dtc2/1
  Gain10_const/1 -> nequ_dtc9/1
  Gain14_const/1 -> nequ_dtc5/1
  Gain12_const/1 -> nequ_dtc7/1
  enb_counter/1 -> enb_counter_eq_15/1, enb_counter_le_15/1
  Gain11_const/1 -> nequ_dtc8/1
  Gain13_const/1 -> nequ_dtc6/1
  Gain5_const/1 -> nequ_dtc14/1
  Gain7_const/1 -> nequ_dtc12/1
  Gain9_const/1 -> nequ_dtc10/1
  Gain4_const/1 -> nequ_dtc15/1
  Gain6_const/1 -> nequ_dtc13/1
  Gain8_const/1 -> nequ_dtc11/1
  in0/1 -> nequ_dtc16/1
  in1/1 -> nequ_dtc17/1
  in2/1 -> nequ_dtc18/1
  demux/15 -> nequ_dtc46/1
  in3/1 -> nequ_dtc19/1
  in8/1 -> nequ_dtc24/1
  in4/1 -> nequ_dtc20/1
  demux/9 -> nequ_dtc40/1
  in5/1 -> nequ_dtc21/1
  demux/6 -> nequ_dtc37/1
  in6/1 -> nequ_dtc22/1
  demux/3 -> nequ_dtc34/1
  in7/1 -> nequ_dtc23/1
  nequ_dtc28/1 -> mux1/13
  in13/1 -> nequ_dtc29/1
  in9/1 -> nequ_dtc25/1
  nequ_dtc27/1 -> mux1/12
  nequ_dtc31/1 -> mux1/16
  in14/1 -> nequ_dtc30/1
  in10/1 -> nequ_dtc26/1
  nequ_dtc30/1 -> mux1/15
  nequ_dtc26/1 -> mux1/11
  in11/1 -> nequ_dtc27/1
  nequ_dtc29/1 -> mux1/14
  in12/1 -> nequ_dtc28/1
  in15/1 -> nequ_dtc31/1
  nequ_dtc4/1 -> mux/5
  nequ_dtc/1 -> mux/1
  nequ_dtc5/1 -> mux/6
  nequ_dtc1/1 -> mux/2
  nequ_dtc2/1 -> mux/3
  nequ_dtc3/1 -> mux/4
  nequ_dtc7/1 -> mux/8
  nequ_dtc9/1 -> mux/10
  nequ_dtc15/1 -> mux/16
  nequ_dtc11/1 -> mux/12
  nequ_dtc13/1 -> mux/14
  nequ_dtc14/1 -> mux/15
  nequ_dtc20/1 -> mux1/5
  nequ_dtc16/1 -> mux1/1
  nequ_dtc17/1 -> mux1/2
  nequ_dtc18/1 -> mux1/3
  nequ_dtc19/1 -> mux1/4
  nequ_dtc25/1 -> mux1/10
  nequ_dtc21/1 -> mux1/6
  nequ_dtc22/1 -> mux1/7
  nequ_dtc23/1 -> mux1/8
  nequ_dtc24/1 -> mux1/9
  enb_counter_le_15/1 -> counter/Enable, tapped_delay/2
  mux/1 -> Serializer_Subnetwork/1(in0)
  mux1/1 -> Serializer_Subnetwork1/1(in0)
  counter/1(out0) -> Serializer_Subnetwork1/2(in1), Serializer_Subnetwork/2(in1)
  Serializer_Subnetwork/1(out0) -> Gain19/1
  Serializer_Subnetwork1/1(out0) -> Gain19/2
  Gain19/1 -> tapped_delay/1
  enb_counter_eq_15/1 -> tapped_delay_outunit_delay/2
  tapped_delay/1 -> tapped_delay_outunit_delay/1
  nequ_dtc45/1 -> out13/1
  tapped_delay_outunit_delay/1 -> demux/1
  demux/1 -> nequ_dtc32/1
  demux/2 -> nequ_dtc33/1
  demux/4 -> nequ_dtc35/1
  demux/5 -> nequ_dtc36/1
  demux/7 -> nequ_dtc38/1
  demux/8 -> nequ_dtc39/1
  demux/10 -> nequ_dtc41/1
  demux/11 -> nequ_dtc42/1
  demux/12 -> nequ_dtc43/1
  demux/13 -> nequ_dtc44/1
  demux/14 -> nequ_dtc45/1
  demux/16 -> nequ_dtc47/1
  nequ_dtc32/1 -> out0/1
  nequ_dtc33/1 -> out1/1
  nequ_dtc34/1 -> out2/1
  nequ_dtc35/1 -> out3/1
  nequ_dtc36/1 -> out4/1
  nequ_dtc37/1 -> out5/1
  nequ_dtc38/1 -> out6/1
  nequ_dtc39/1 -> out7/1
  nequ_dtc40/1 -> out8/1
  nequ_dtc41/1 -> out9/1
  nequ_dtc42/1 -> out10/1
  nequ_dtc43/1 -> out11/1
  nequ_dtc44/1 -> out12/1
  nequ_dtc46/1 -> out14/1
  nequ_dtc47/1 -> out15/1

== system gm_HFMA_4B_1_5_9_13/Subsystem/crp_temp_shared6 ==
  in0 : Inport  OutDataTypeStr=fixdt(1,16,15,'DataTypeOverride', 'Off')  PortDimensions=1  SampleTime=1.953125e-06
  in1 : Inport  Port=2  OutDataTypeStr=fixdt(1,16,15,'DataTypeOverride', 'Off')  PortDimensions=1  SampleTime=1.953125e-06
  in2 : Inport  Port=3  OutDataTypeStr=fixdt(1,16,15,'DataTypeOverride', 'Off')  PortDimensions=1  SampleTime=1.953125e-06
  in3 : Inport  Port=4  OutDataTypeStr=fixdt(1,16,15,'DataTypeOverride', 'Off')  PortDimensions=1  SampleTime=1.953125e-06
  enb_counter : Inport  Port=5  OutDataTypeStr=fixdt(0,6,0,'DataTypeOverride', 'Off')  PortDimensions=1  SampleTime=1.953125e-06
  Gain1_const : Constant  Value=-0.003899991512298583984375  OutDataTypeStr=fixdt(1, 18, 25)  SampleTime=1.953125e-06
  Gain2_const : Constant  Value=0.001299999654293060302734375  OutDataTypeStr=fixdt(0, 18, 27)  SampleTime=1.953125e-06
  Gain3 : Product  Inputs=**  OutDataTypeStr=fixdt(1, 35, 0)  SampleTime=1.953125e-06
  Gain3_const : Constant  Value=-0.0132000446319580078125  OutDataTypeStr=fixdt(1, 18, 23)  SampleTime=1.953125e-06
  Gain_const : Constant  Value=0.0005999989807605743408203125  OutDataTypeStr=fixdt(0, 18, 28)  SampleTime=1.953125e-06
  Serializer_Subnetwork : Subsystem
  Serializer_Subnetwork1 : Subsystem
  counter : Subsystem
  demux : Demux
  enb_counter_eq_3 : simulink/Logic and Bit Operations/Compare To Constant  relop===  const=3  OutDataTypeStr=boolean
  enb_counter_le_3 : simulink/Logic and Bit Operations/Compare To Constant  relop=<=  const=3  OutDataTypeStr=boolean
  mux : Mux
  mux1 : Mux
  nequ_dtc{,1..3} (4 alike) : DataTypeConversion  OutDataTypeStr=fixdt(1, 19, 0)  ConvertRealWorld=Stored Integer (SI)  SampleTime=1.953125e-06  SaturateOnIntegerOverflow=off  RndMeth=Floor
  nequ_dtc10 : DataTypeConversion  OutDataTypeStr=fixdt(1, 34, 40)  ConvertRealWorld=Stored Integer (SI)  SampleTime=1.953125e-06  SaturateOnIntegerOverflow=off  RndMeth=Floor
  nequ_dtc11 : DataTypeConversion  OutDataTypeStr=fixdt(1, 34, 43)  ConvertRealWorld=Stored Integer (SI)  SampleTime=1.953125e-06  SaturateOnIntegerOverflow=off  RndMeth=Floor
  nequ_dtc{4..7} (4 alike) : DataTypeConversion  OutDataTypeStr=fixdt(1, 17, 0)  ConvertRealWorld=Stored Integer (SI)  SampleTime=1.953125e-06  SaturateOnIntegerOverflow=off  RndMeth=Floor
  nequ_dtc8 : DataTypeConversion  OutDataTypeStr=fixdt(1, 34, 38)  ConvertRealWorld=Stored Integer (SI)  SampleTime=1.953125e-06  SaturateOnIntegerOverflow=off  RndMeth=Floor
  nequ_dtc9 : DataTypeConversion  OutDataTypeStr=fixdt(1, 34, 42)  ConvertRealWorld=Stored Integer (SI)  SampleTime=1.953125e-06  SaturateOnIntegerOverflow=off  RndMeth=Floor
  tapped_delay : hdlsllib/Discrete/Tapped Delay Enabled Synchronous  vinit=0  samptime=-1  NumDelays=3  DelayOrder=Oldest  includeCurrent=on
  tapped_delay_outunit_delay : simulink_need_slupdate/Unit Delay Enabled  vinit=0.0  tsamp=-1
  out0 : Outport  OutDataTypeStr=fixdt(1,34,38,'DataTypeOverride', 'Off')  PortDimensions=1  SampleTime=1.953125e-06
  out1 : Outport  Port=2  OutDataTypeStr=fixdt(1,34,42,'DataTypeOverride', 'Off')  PortDimensions=1  SampleTime=1.953125e-06
  out2 : Outport  Port=3  OutDataTypeStr=fixdt(1,34,40,'DataTypeOverride', 'Off')  PortDimensions=1  SampleTime=1.953125e-06
  out3 : Outport  Port=4  OutDataTypeStr=fixdt(1,34,43,'DataTypeOverride', 'Off')  PortDimensions=1  SampleTime=1.953125e-06
  wires:
  Gain3/1 -> tapped_delay/1
  Gain2_const/1 -> nequ_dtc1/1
  Gain_const/1 -> nequ_dtc3/1
  Gain3_const/1 -> nequ_dtc/1
  Gain1_const/1 -> nequ_dtc2/1
  in1/1 -> nequ_dtc5/1
  in0/1 -> nequ_dtc4/1
  in3/1 -> nequ_dtc7/1
  Serializer_Subnetwork1/1(out0) -> Gain3/2
  in2/1 -> nequ_dtc6/1
  enb_counter/1 -> enb_counter_le_3/1, enb_counter_eq_3/1
  nequ_dtc/1 -> mux/1
  nequ_dtc1/1 -> mux/2
  nequ_dtc2/1 -> mux/3
  nequ_dtc5/1 -> mux1/2
  nequ_dtc3/1 -> mux/4
  Serializer_Subnetwork/1(out0) -> Gain3/1
  nequ_dtc4/1 -> mux1/1
  nequ_dtc8/1 -> out0/1
  demux/3 -> nequ_dtc10/1
  nequ_dtc6/1 -> mux1/3
  nequ_dtc9/1 -> out1/1
  demux/2 -> nequ_dtc9/1
  nequ_dtc7/1 -> mux1/4
  enb_counter_le_3/1 -> counter/Enable, tapped_delay/2
  mux/1 -> Serializer_Subnetwork/1(in0)
  mux1/1 -> Serializer_Subnetwork1/1(in0)
  counter/1(out0) -> Serializer_Subnetwork1/2(in1), Serializer_Subnetwork/2(in1)
  enb_counter_eq_3/1 -> tapped_delay_outunit_delay/2
  tapped_delay/1 -> tapped_delay_outunit_delay/1
  nequ_dtc11/1 -> out3/1
  tapped_delay_outunit_delay/1 -> demux/1
  demux/1 -> nequ_dtc8/1
  demux/4 -> nequ_dtc11/1
  nequ_dtc10/1 -> out2/1
